simulink model "ToyChart"  (R2023b)
settings: Solver=VariableStepAuto  StartTime=0.0  StopTime=10.0  RelTol=1e-3
settings Model: Creator=na  LastModifiedBy=na

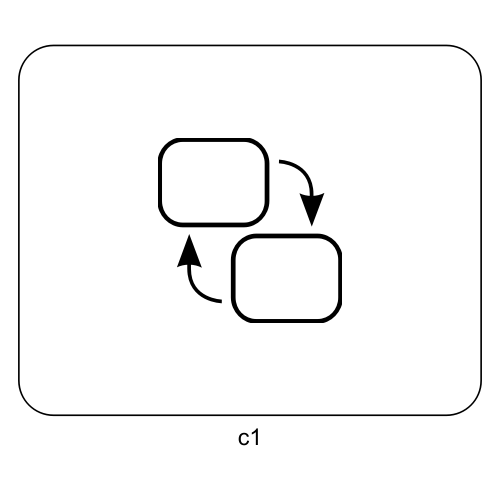
[thumbnail: Simulink's stored preview of the top-level diagram]
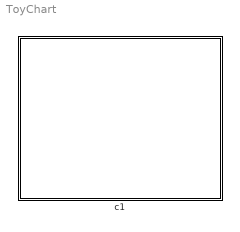
== system ToyChart ==
  c1 : Stateflow chart  TreatAsAtomicUnit=on

== stateflow chart ToyChart/c1 ==
  state On
  state Off
  On -> Off : timeout
